simulink model "flickertesting"  (R2024a)
settings: Solver=VariableStepAuto  StartTime=0.0  StopTime=1  RelTol=1e-3
libraries: simulink_extras x1, cstblocks x1, dspobslib x1
settings Model: Creator=SHASHANK DADURIA  LastModifiedBy=srima

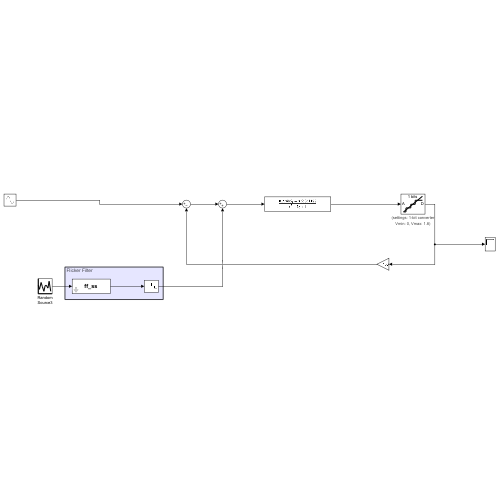
[thumbnail: Simulink's stored preview of the top-level diagram]
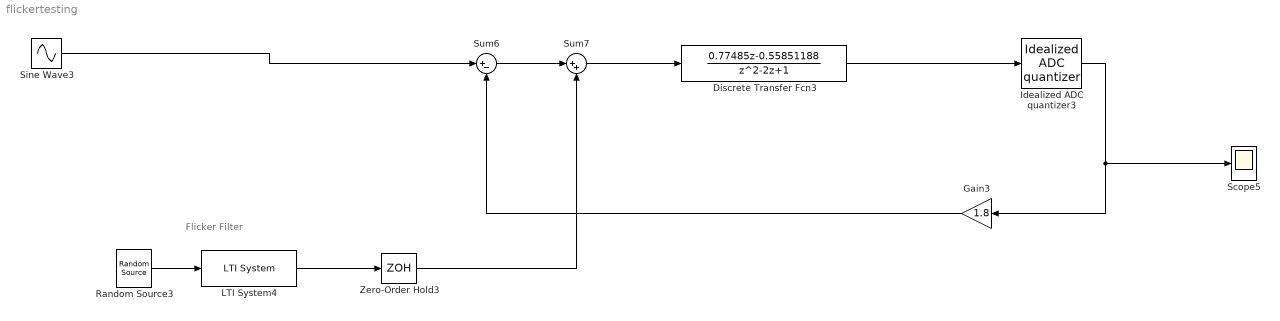
== system flickertesting ==
  note: Flicker Filter
  Discrete Transfer Fcn3 : DiscreteTransferFcn  Numerator=[0.77485 -0.55851188]  Denominator=[1 -2 1]
  Gain3 : Gain  Gain=1.8
  Idealized ADC quantizer3 : simulink_extras/Additional Discrete/Idealized ADC quantizer  NumberOfConverterBits=1  Vmin=0  Vmax=1.8  OutputDataType=int32  OutputNegativeValues=off
  LTI System4 : cstblocks/LTI System  sys=ff_ss  IC=[]  PadeOrder=0
  Random Source3 : dspobslib/Random Source  SrcType=Gaussian  NormMethod=Ziggurat  CltLength=12  MinVal=0  MaxVal=1  MeanVal=0  VarVal=1e-20  RepMode=Not repeatable  rawSeed=1  IsInherit=off  SampMode=Discrete  SampTime=1/(2000*2048)  SampFrame=1  DataType=Double  OutComplex=Real  OutputFrames=off
  Scope5 : Scope
  Sine Wave3 : Sin  Amplitude=0.6  Bias=0.9  Frequency=((2000*1024)*127*2*2*pi)/(32768*32)  SampleTime=1/(2000*2048)
  Sum6 : Sum  Inputs=|+-
  Sum7 : Sum  Inputs=|++
  Zero-Order Hold3 : ZeroOrderHold  SampleTime=1/(2000*2048)
  wires:
  Discrete Transfer Fcn3/1 -> Idealized ADC quantizer3/1
  LTI System4/1 -> Zero-Order Hold3/1
  Sum6/1 -> Sum7/1
  Sum7/1 -> Discrete Transfer Fcn3/1
  Zero-Order Hold3/1 -> Sum7/2
  Gain3/1 -> Sum6/2
  Idealized ADC quantizer3/1 -> Scope5/1, Gain3/1
  Random Source3/1 -> LTI System4/1
  Sine Wave3/1 -> Sum6/1
